simulink model "s_c_nbe_m32k"  (R2018a)
settings: Solver=VariableStepDiscrete  StartTime=0.0  StopTime=1000  RelTol=1e-3
undefined symbols (not defined in the file): fft_stages, n_taps, output_bits, pfb_coeff_gen_calc, xengbits
libraries: xbsIndex_r4 x23714, casper_library_misc x17, xps_library x4, casper_library_scopes x4, xbsReplacements_r4 x4
(part 25 of 171)

== system s_c_nbe_m32k/quant1 ==
  sync_in : Inport
  din : Inport  Port=2
  en : Inport  Port=3
  coeffs : Inport  Port=4
  Delay1 : xbsIndex_r4/Delay  rst=off  infoeditControl=Selection of Reset will increase slice count due to use of real FFs and instead of SRLs  en=off  latency=conv_latency  reg_retiming=on  dbl_ovrd=off  block_type=delay
  Delay2 : xbsIndex_r4/Delay  rst=off  infoeditControl=Selection of Reset will increase slice count due to use of real FFs and instead of SRLs  en=off  latency=conv_latency  reg_retiming=on  dbl_ovrd=off  block_type=delay
  Delay3 : xbsIndex_r4/Delay  rst=off  infoeditControl=Selection of Reset will increase slice count due to use of real FFs and instead of SRLs  en=off  latency=2  reg_retiming=on  dbl_ovrd=off  block_type=delay
  Delay4 : xbsIndex_r4/Delay  rst=off  infoeditControl=Selection of Reset will increase slice count due to use of real FFs and instead of SRLs  en=off  latency=2  reg_retiming=on  dbl_ovrd=off  block_type=delay
  Delay6 : xbsIndex_r4/Delay  rst=off  infoeditControl=Selection of Reset will increase slice count due to use of real FFs and instead of SRLs  en=off  latency=2  reg_retiming=on  dbl_ovrd=off  block_type=delay
  bus_constant : Subsystem  mask(bus_constant){values=repmat(-1+1/(2^dout_bin_pt), 1, 8), n_bits=dout_bit_width, bin_pts=dout_bin_pt, types=[1]}
      mask prompts: n_bits "bit widths"; bin_pts "binary points"; types "data type"
      mask help: Combine constants into a bus
      mask init:
      | bus_constant_init(gcb, ...
      |     'values', values, ...
      |     'n_bits', n_bits, ...
      |     'bin_pts', bin_pts, ...
      |     'types', types);
  bus_constant1 : Subsystem  mask(bus_constant){values=repmat(-1+1/(2^dout_bin_pt), 1, 8), n_bits=din_bit_width+coeff_bit_width+1, bin_pts=din_bin_pt+coeff_bin_pt, types=[1]}
      mask prompts: n_bits "bit widths"; bin_pts "binary points"; types "data type"
      mask help: Combine constants into a bus
      mask init:
      | bus_constant_init(gcb, ...
      |     'values', values, ...
      |     'n_bits', n_bits, ...
      |     'bin_pts', bin_pts, ...
      |     'types', types);
  bus_convert : Subsystem  Tag=cmac_delinked  mask(bus_convert){n_bits_in=repmat(din_bit_width+coeff_bit_width+1, 1, 8), bin_pt_in=din_bin_pt+coeff_bin_pt, cmplx=off, n_bits_out=8, bin_pt_out=7, quantization=2, overflow=1, csp_latency=conv_latency, of=on, misc=off}
      mask prompts: n_bits_in "input bit widths"; bin_pt_in "input binary points"; cmplx "input complex"; n_bits_out "output bit widths"; bin_pt_out "output binary points"; quantization "quantization strategy (Truncate=0, Round  (unbiased: +/- Inf)=1, Round (unbiased: Even Values)=2)"; overflow "overflow strategy (Wrap=0, Saturate=1, Flag as error=2)"; csp_latency "latency"; of "overflow indication"; misc "misc support"
      mask help: Convert components of busses
      mask init: same as s_c_nbe_m32k/cwg_cos/bus_convert
  bus_create : Subsystem  mask(bus_create){inputNum=2}
      mask prompts: inputNum "Number of inputs:"
      mask init:
      | bus_create_init(gcb,...
      |     'inputNum', inputNum);
  bus_expand1 : Subsystem  mask(bus_expand){mode=divisions of equal size, outputNum=2, outputWidth=1, outputBinaryPt=0, outputArithmeticType=2, show_format=off, outputToWorkspace=off, variablePrefix=out, outputToModelAsWell=on}
      mask prompts: outputNum "Number of outputs:"; outputWidth "Output width:"; outputBinaryPt "Output binary point position:"; outputArithmeticType "Output arithmetic type (ufix=0, fix=1, bool=2):"; show_format "Print format string?"; outputToWorkspace "Output to workspace?"; variablePrefix "Variable name prefix:"; outputToModelAsWell "Output to model as well?"
      mask help:
      | Expands a 'bus' made using a bus_create or Xilinx
      | concat block.
      | The input will be divided into the specified number
      | of outputs with the specified arithmetic types.
      | Divisions are made from most significant bit.
      mask init: same as s_c_nbe_m32k/bus_expand1
      settings: AttributesFormatString=2 outputs
      mask TypeOptions mode: divisions of equal size | divisions of arbitrary size
      mask Callback mode: bus_expand_callback();
      mask Callback outputWidth: bus_expand_callback();
      mask Callback outputToWorkspace: bus_expand_callback();
  bus_mult : Subsystem  mask(bus_mult){n_bits_a=repmat(din_bit_width, 1, 4), bin_pt_a=din_bin_pt, type_a=1, cmplx_a=on, n_bits_b=repmat(coeff_bit_width, 1, 4), bin_pt_b=coeff_bin_pt, type_b=1, cmplx_b=on, n_bits_out=din_bit_width+coeff_bit_width+1, bin_pt_out=din_bin_pt+coeff_bin_pt, type_out=1, quantization=0, overflow=0, mult_latency=3, add_latency=1, conv_latency=0, max_fanout=1, fan_latency=1, multiplier_implementation=behavioral HDL, misc=on}
      mask prompts: n_bits_a "a input bit widths"; bin_pt_a "a input binary points"; type_a "a input type (Unsigned=0, Signed=1)"; cmplx_a "a input complex"; n_bits_b "b input bit widths"; bin_pt_b "b input binary points"; type_b "b input type (Unsigned=0, Signed=1)"; cmplx_b "b input complex"; n_bits_out "output bit widths"; bin_pt_out "output binary points"; type_out "output type (Unsigned=0, Signed=1)"; quantization "quantization strategy (Truncate=0, Round  (unbiased: +/- Inf)=1)"; overflow "overflow strategy (Wrap=0, Saturate=1, Flag as error=2)"; mult_latency "multiplier latency"; add_latency "adder latency"; conv_latency "convert latency"; max_fanout "limit fanout to ?"; fan_latency "fanout register latency"; multiplier_implementation "multiplier implementation"; misc "misc support"
      mask help: Multiply components of two busses
      mask init: same as s_c_nbe_m32k/quant0/bus_mult
      mask TypeOptions multiplier_implementation: behavioral HDL | standard core | embedded multiplier core
  bus_mux : Subsystem  mask(bus_mux){n_inputs=2, n_bits=repmat(8, 1, 8), mux_latency=2, cmplx=off, misc=off}
      mask prompts: n_inputs "number of inputs"; n_bits "input bit widths"; mux_latency "mux latency"; cmplx "complex data"; misc "misc support"
      mask help: Mux components of bus
      mask init:
      | bus_mux_init(gcb, ...
      |     'n_inputs', n_inputs, ...
      |     'n_bits', n_bits, ...
      |     'cmplx', cmplx, ...
      |     'misc', misc, ...
      |     'mux_latency', mux_latency);
  bus_relational : Subsystem  Tag=cmac_delinked  mask(bus_relational){n_bits_a=repmat(din_bit_width+coeff_bit_width+1, 1, 8), bin_pt_a=din_bin_pt+coeff_bin_pt, type_a=1, n_bits_b=repmat(din_bit_width+coeff_bit_width+1, 1, 8), bin_pt_b=din_bin_pt+coeff_bin_pt, type_b=1, en=off, misc=off, mode=a<b, csp_latency=conv_latency}
      mask prompts: n_bits_a "a input bit widths"; bin_pt_a "a input binary points"; type_a "a input type (Unsigned=0, Signed=1)"; n_bits_b "b input bit widths"; bin_pt_b "b input binary points"; type_b "b input type (Unsigned=0, Signed=1)"; en "en port"; misc "misc support"; mode "comparison:"; csp_latency "latency"
      mask help: Find the relational product of two busses
      mask init: same as s_c_nbe_m32k/quant0/bus_relational
      mask TypeOptions mode: a=b | a!=b | a<b | a>b | a<=b | a>=b
  pipeline1 : Subsystem  Tag=cmac_delinked  mask(pipeline){csp_latency=2}
      mask prompts: csp_latency "Latency"
      mask help:
      | An explicitly laid-out delay line to avoid mapping to SRL16s
      | for use in pipelining to help achieve timing closure.
      mask init:
      | pipeline_init(gcb,'latency',csp_latency);
      settings: AttributesFormatString=Latency = %<latency>
      mask Display:
      | port_label('input', 1, 'd');
      | port_label('output', 1, 'q');
      | disp(['Z^-', num2str(csp_latency)]);
  pipeline10 : Subsystem  Tag=cmac_delinked  mask(pipeline){csp_latency=2}
      mask prompts: csp_latency "Latency"
      mask help:
      | An explicitly laid-out delay line to avoid mapping to SRL16s
      | for use in pipelining to help achieve timing closure.
      mask init:
      | pipeline_init(gcb,'latency',csp_latency);
      settings: AttributesFormatString=Latency = %<latency>
      mask Display:
      | port_label('input', 1, 'd');
      | port_label('output', 1, 'q');
      | disp(['Z^-', num2str(csp_latency)]);
  pipeline2 : Subsystem  Tag=cmac_delinked  mask(pipeline){csp_latency=2}
      mask prompts: csp_latency "Latency"
      mask help:
      | An explicitly laid-out delay line to avoid mapping to SRL16s
      | for use in pipelining to help achieve timing closure.
      mask init:
      | pipeline_init(gcb,'latency',csp_latency);
      settings: AttributesFormatString=Latency = %<latency>
      mask Display:
      | port_label('input', 1, 'd');
      | port_label('output', 1, 'q');
      | disp(['Z^-', num2str(csp_latency)]);
  pipeline3 : Subsystem  Tag=cmac_delinked  mask(pipeline){csp_latency=2}
      mask prompts: csp_latency "Latency"
      mask help:
      | An explicitly laid-out delay line to avoid mapping to SRL16s
      | for use in pipelining to help achieve timing closure.
      mask init:
      | pipeline_init(gcb,'latency',csp_latency);
      settings: AttributesFormatString=Latency = %<latency>
      mask Display:
      | port_label('input', 1, 'd');
      | port_label('output', 1, 'q');
      | disp(['Z^-', num2str(csp_latency)]);
  pipeline4 : Subsystem  Tag=cmac_delinked  mask(pipeline){csp_latency=2}
      mask prompts: csp_latency "Latency"
      mask help:
      | An explicitly laid-out delay line to avoid mapping to SRL16s
      | for use in pipelining to help achieve timing closure.
      mask init:
      | pipeline_init(gcb,'latency',csp_latency);
      settings: AttributesFormatString=Latency = %<latency>
      mask Display:
      | port_label('input', 1, 'd');
      | port_label('output', 1, 'q');
      | disp(['Z^-', num2str(csp_latency)]);
  pipeline45 : Subsystem  Tag=cmac_delinked  mask(pipeline){csp_latency=2}
      mask prompts: csp_latency "Latency"
      mask help:
      | An explicitly laid-out delay line to avoid mapping to SRL16s
      | for use in pipelining to help achieve timing closure.
      mask init:
      | pipeline_init(gcb,'latency',csp_latency);
      settings: AttributesFormatString=Latency = %<latency>
      mask Display:
      | port_label('input', 1, 'd');
      | port_label('output', 1, 'q');
      | disp(['Z^-', num2str(csp_latency)]);
  pipeline5 : Subsystem  Tag=cmac_delinked  mask(pipeline){csp_latency=2}
      mask prompts: csp_latency "Latency"
      mask help:
      | An explicitly laid-out delay line to avoid mapping to SRL16s
      | for use in pipelining to help achieve timing closure.
      mask init:
      | pipeline_init(gcb,'latency',csp_latency);
      settings: AttributesFormatString=Latency = %<latency>
      mask Display:
      | port_label('input', 1, 'd');
      | port_label('output', 1, 'q');
      | disp(['Z^-', num2str(csp_latency)]);
  pipeline6 : Subsystem  Tag=cmac_delinked  mask(pipeline){csp_latency=2}
      mask prompts: csp_latency "Latency"
      mask help:
      | An explicitly laid-out delay line to avoid mapping to SRL16s
      | for use in pipelining to help achieve timing closure.
      mask init:
      | pipeline_init(gcb,'latency',csp_latency);
      settings: AttributesFormatString=Latency = %<latency>
      mask Display:
      | port_label('input', 1, 'd');
      | port_label('output', 1, 'q');
      | disp(['Z^-', num2str(csp_latency)]);
  pipeline7 : Subsystem  Tag=cmac_delinked  mask(pipeline){csp_latency=2}
      mask prompts: csp_latency "Latency"
      mask help:
      | An explicitly laid-out delay line to avoid mapping to SRL16s
      | for use in pipelining to help achieve timing closure.
      mask init:
      | pipeline_init(gcb,'latency',csp_latency);
      settings: AttributesFormatString=Latency = %<latency>
      mask Display:
      | port_label('input', 1, 'd');
      | port_label('output', 1, 'q');
      | disp(['Z^-', num2str(csp_latency)]);
  pipeline8 : Subsystem  Tag=cmac_delinked  mask(pipeline){csp_latency=2}
      mask prompts: csp_latency "Latency"
      mask help:
      | An explicitly laid-out delay line to avoid mapping to SRL16s
      | for use in pipelining to help achieve timing closure.
      mask init:
      | pipeline_init(gcb,'latency',csp_latency);
      settings: AttributesFormatString=Latency = %<latency>
      mask Display:
      | port_label('input', 1, 'd');
      | port_label('output', 1, 'q');
      | disp(['Z^-', num2str(csp_latency)]);
  pipeline9 : Subsystem  Tag=cmac_delinked  mask(pipeline){csp_latency=2}
      mask prompts: csp_latency "Latency"
      mask help:
      | An explicitly laid-out delay line to avoid mapping to SRL16s
      | for use in pipelining to help achieve timing closure.
      mask init:
      | pipeline_init(gcb,'latency',csp_latency);
      settings: AttributesFormatString=Latency = %<latency>
      mask Display:
      | port_label('input', 1, 'd');
      | port_label('output', 1, 'q');
      | disp(['Z^-', num2str(csp_latency)]);
  sync_out : Outport
  dout : Outport  Port=2
  dvalid : Outport  Port=3
  of : Outport  Port=4
  wires:
  pipeline10/1(q) -> dvalid/1
  pipeline9/1(q) -> sync_out/1
  pipeline8/1(q) -> of/1
  pipeline7/1(q) -> dout/1
  pipeline6/1(q) -> bus_expand1/1(bus_in)
  pipeline5/1(q) -> bus_convert/1(din)
  pipeline4/1(q) -> bus_relational/1(a)
  pipeline3/1(q) -> bus_create/2(in2)
  pipeline2/1(q) -> bus_create/1(in1)
  pipeline1/1(q) -> bus_mult/2(b)
  pipeline45/1(q) -> bus_mult/1(a)
  Delay4/1 -> pipeline8/1(d)
  bus_convert/2(overflow) -> Delay4/1
  bus_mux/1(out) -> pipeline7/1(d)
  bus_constant1/1(dout) -> bus_relational/2(b)
  bus_constant/1(dout) -> bus_mux/3(d1)
  bus_convert/1(dout) -> bus_mux/2(d0)
  bus_relational/1(a<b) -> bus_mux/1(sel)
  Delay3/1 -> pipeline10/1(d)
  bus_expand1/2(lsb_out1) -> Delay1/1
  Delay1/1 -> Delay3/1
  bus_expand1/1(msb_out2) -> Delay2/1
  bus_mult/2(misco) -> pipeline6/1(d)
  bus_mult/1(a*b) -> pipeline4/1(d), pipeline5/1(d)
  bus_create/1(bus_out) -> bus_mult/3(misci)
  en/1 -> pipeline3/1(d)
  sync_in/1 -> pipeline2/1(d)
  coeffs/1 -> pipeline1/1(d)
  din/1 -> pipeline45/1(d)
  Delay6/1 -> pipeline9/1(d)
  Delay2/1 -> Delay6/1

== system s_c_nbe_m32k/quant_pwr0 ==
  out_reg : Inport
  assert_reg : xbsIndex_r4/Assert  assert_type=on  type_source=Explicitly  gui_display_data_type=Fixed-point  arith_type=Unsigned  n_bits=32  bin_pt=31  preci_type=Single  exp_width=8  frac_width=24  assert_rate=off  rate_source=Explicitly  period=1  output_port=on  block_type=assert
  cast_gw : xbsIndex_r4/Convert  gui_display_data_type=Fixed-point  arith_type=Unsigned  n_bits=32  bin_pt=0  float_type=Single  exp_bits=8  fraction_bits=24  quantization=Truncate  overflow=Wrap  en=off  latency=1  pipeline=off  dbl_ovrd=off  block_type=convert
  io_delay : xbsIndex_r4/Delay  rst=off  infoeditControl=Selection of Reset will increase slice count due to use of real FFs and instead of SRLs  en=off  latency=0  reg_retiming=on  dbl_ovrd=off  block_type=delay
  reint1 : xbsIndex_r4/Reinterpret  force_arith_type=on  arith_type=Unsigned  force_bin_pt=on  bin_pt=0  block_type=reinterpret
  s_c_nbe_m32k_v9_quant_pwr0_user_data_in : xbsIndex_r4/Gateway Out  inherit_from_input=off  hdl_port=on  rows=1  columns=1  UseAsDAC=off  DACChannel='1'  interface=None  automatic_assignment=on  address_offset=hex2dec('00')  intf_name=''  intf_description=''  timing_constraint=None  locs_specified=off  LOCs={}  io_standard={}  block_type=gatewayout
  sim_out : Terminator
  wires:
  io_delay/1 -> cast_gw/1
  cast_gw/1 -> s_c_nbe_m32k_v9_quant_pwr0_user_data_in/1
  s_c_nbe_m32k_v9_quant_pwr0_user_data_in/1 -> sim_out/1
  out_reg/1 -> assert_reg/1
  assert_reg/1 -> reint1/1
  reint1/1 -> io_delay/1

== system s_c_nbe_m32k/quant_pwr1 ==
  out_reg : Inport
  assert_reg : xbsIndex_r4/Assert  assert_type=on  type_source=Explicitly  gui_display_data_type=Fixed-point  arith_type=Unsigned  n_bits=32  bin_pt=31  preci_type=Single  exp_width=8  frac_width=24  assert_rate=off  rate_source=Explicitly  period=1  output_port=on  block_type=assert
  cast_gw : xbsIndex_r4/Convert  gui_display_data_type=Fixed-point  arith_type=Unsigned  n_bits=32  bin_pt=0  float_type=Single  exp_bits=8  fraction_bits=24  quantization=Truncate  overflow=Wrap  en=off  latency=1  pipeline=off  dbl_ovrd=off  block_type=convert
  io_delay : xbsIndex_r4/Delay  rst=off  infoeditControl=Selection of Reset will increase slice count due to use of real FFs and instead of SRLs  en=off  latency=0  reg_retiming=on  dbl_ovrd=off  block_type=delay
  reint1 : xbsIndex_r4/Reinterpret  force_arith_type=on  arith_type=Unsigned  force_bin_pt=on  bin_pt=0  block_type=reinterpret
  s_c_nbe_m32k_v9_quant_pwr1_user_data_in : xbsIndex_r4/Gateway Out  inherit_from_input=off  hdl_port=on  rows=1  columns=1  UseAsDAC=off  DACChannel='1'  interface=None  automatic_assignment=on  address_offset=hex2dec('00')  intf_name=''  intf_description=''  timing_constraint=None  locs_specified=off  LOCs={}  io_standard={}  block_type=gatewayout
  sim_out : Terminator
  wires:
  io_delay/1 -> cast_gw/1
  cast_gw/1 -> s_c_nbe_m32k_v9_quant_pwr1_user_data_in/1
  s_c_nbe_m32k_v9_quant_pwr1_user_data_in/1 -> sim_out/1
  out_reg/1 -> assert_reg/1
  assert_reg/1 -> reint1/1
  reint1/1 -> io_delay/1

== system s_c_nbe_m32k/quant_snap_ctrl ==
  sim_1 : Inport
  sim_2 : Inport  Port=2
  convert1_1 : DataTypeConversion  OutDataTypeStr=fixdt('ufix1_En0')  LockScale=on
  convert1_2 : DataTypeConversion  OutDataTypeStr=fixdt('ufix31_En0')  LockScale=on
  convert2_1 : DataTypeConversion  OutDataTypeStr=fixdt('ufix1_En0')  ConvertRealWorld=Stored Integer (SI)  LockScale=on
  convert2_2 : DataTypeConversion  OutDataTypeStr=fixdt('ufix31_En0')  ConvertRealWorld=Stored Integer (SI)  LockScale=on
  gain_1 : Gain  Gain=2147483648
  gain_2 : Gain
  io_delay : xbsIndex_r4/Delay  rst=off  infoeditControl=Selection of Reset will increase slice count due to use of real FFs and instead of SRLs  en=off  latency=0  reg_retiming=on  dbl_ovrd=off  block_type=delay
  reint2 : xbsIndex_r4/Reinterpret  force_arith_type=on  arith_type=Unsigned  force_bin_pt=on  bin_pt=0  block_type=reinterpret
  s_c_nbe_m32k_v9_quant_snap_ctrl_user_data_out : xbsIndex_r4/Gateway In  gui_display_data_type=Fixed-point  arith_type=Unsigned  n_bits=32  bin_pt=0  preci_type=Single  exp_width=8  frac_width=24  rows=1  columns=1  quantization="Round  (unbiased: +/- Inf)"  overflow=Saturate  period=1  UseAsADC=off  ADCChannel='1'  interface=None  automatic_assignment=on  address_offset=hex2dec('00')  intf_name=''  intf_description=''  default_value=0  timing_constraint=None  locs_specified=off  LOCs={}  io_standard={}  inherit_from_input=off  hdl_port=on  dbl_ovrd=off  block_type=gatewayin
  sim_add : Sum  OutDataTypeStr=uint32
  slice_channel_select : xbsIndex_r4/Slice  nbits=31  boolean_output=off  mode=Lower Bit Location + Width  bit1=0  base1=MSB of Input  bit0=0  base0=LSB of Input  dbl_ovrd=off  block_type=slice
  slice_single_channel : xbsIndex_r4/Slice  nbits=1  boolean_output=on  mode=Lower Bit Location + Width  bit1=0  base1=MSB of Input  bit0=31  base0=LSB of Input  dbl_ovrd=off  block_type=slice
  in_single_channel : Outport
  in_channel_select : Outport  Port=2
  wires:
  s_c_nbe_m32k_v9_quant_snap_ctrl_user_data_out/1 -> io_delay/1
  sim_add/1 -> s_c_nbe_m32k_v9_quant_snap_ctrl_user_data_out/1
  sim_1/1 -> convert1_1/1
  convert1_1/1 -> convert2_1/1
  convert2_1/1 -> gain_1/1
  gain_1/1 -> sim_add/1
  io_delay/1 -> slice_single_channel/1, slice_channel_select/1
  slice_single_channel/1 -> in_single_channel/1
  sim_2/1 -> convert1_2/1
  convert1_2/1 -> convert2_2/1
  convert2_2/1 -> gain_2/1
  gain_2/1 -> sim_add/2
  slice_channel_select/1 -> reint2/1
  reint2/1 -> in_channel_select/1

== system s_c_nbe_m32k/quant_snap_filter0 ==
  note: This block filters out a single channel
      | from the quantiser so that if you want to get
      | a time-series of them in the snap instead of
      | a spectrum, you can do so.
  sync_in : Inport
  data_valid_in : Inport  Port=2
  data_in : Inport  Port=3
  packet_sync_in : Inport  Port=4
  single_channel_enable : Inport  Port=5
  channel_select : Inport  Port=6
  Counter : xbsIndex_r4/Counter  cnt_type=Free Running  cnt_to=4095  operation=Up  start_count=0  cnt_by_val=1  arith_type=Unsigned  n_bits=fft_stages - 3  bin_pt=0  load_pin=off  rst=on  en=on  explicit_period=on  period=1  use_behavioral_HDL=off  implementation=Fabric  dbl_ovrd=off  block_type=counter
  Delay : xbsIndex_r4/Delay  rst=off  infoeditControl=Selection of Reset will increase slice count due to use of real FFs and instead of SRLs  en=off  latency=1  reg_retiming=off  dbl_ovrd=off  block_type=delay
      settings: infoedit=Hardware notes: A delay line is a chain, each link of which is an SRL16 or SRL32 followed by a flip-flop.
  Delay1 : xbsIndex_r4/Delay  rst=off  infoeditControl=Selection of Reset will increase slice count due to use of real FFs and instead of SRLs  en=off  latency=1  reg_retiming=off  dbl_ovrd=off  block_type=delay
      settings: infoedit=Hardware notes: A delay line is a chain, each link of which is an SRL16 or SRL32 followed by a flip-flop.
  Mux1 : xbsIndex_r4/Mux  inputs=2  en=off  latency=3  precision=Full  arith_type=Unsigned  n_bits=16  bin_pt=14  quantization=Truncate  overflow=Wrap  dbl_ovrd=off  block_type=mux
  Relational : xbsIndex_r4/Relational  mode=a=b  op_type=Bool  en=off  latency=0  dbl_ovrd=off  block_type=relational
  data_valid_out : Outport
  data_out : Outport  Port=2
  packet_sync_out : Outport  Port=3
  wires:
  [packet_sync] -> Delay1/1
  Delay/1 -> data_out/1
  data_valid_in/1 -> [data_valid]
  [sync_in] -> Counter/1
  Mux1/1 -> data_valid_out/1
  data_in/1 -> [data]
  [data_valid] -> Mux1/2
  Relational/1 -> [selected_channel_active]
  Counter/1 -> Relational/1
  sync_in/1 -> [sync_in]
  [selected_channel_active] -> Mux1/3
  packet_sync_in/1 -> [packet_sync]
  [data] -> Delay/1
  [channel_select] -> Relational/2
  Delay1/1 -> packet_sync_out/1
  single_channel_enable/1 -> [single_channel_enable]
  [data_valid] -> Counter/2
  [single_channel_enable] -> Mux1/1
  channel_select/1 -> [channel_select]

== system s_c_nbe_m32k/quant_snap_filter1 ==
  note: This block filters out a single channel
      | from the quantiser so that if you want to get
      | a time-series of them in the snap instead of
      | a spectrum, you can do so.
  sync_in : Inport
  data_valid_in : Inport  Port=2
  data_in : Inport  Port=3
  packet_sync_in : Inport  Port=4
  single_channel_enable : Inport  Port=5
  channel_select : Inport  Port=6
  Counter : xbsIndex_r4/Counter  cnt_type=Free Running  cnt_to=4095  operation=Up  start_count=0  cnt_by_val=1  arith_type=Unsigned  n_bits=fft_stages - 3  bin_pt=0  load_pin=off  rst=on  en=on  explicit_period=on  period=1  use_behavioral_HDL=off  implementation=Fabric  dbl_ovrd=off  block_type=counter
  Delay : xbsIndex_r4/Delay  rst=off  infoeditControl=Selection of Reset will increase slice count due to use of real FFs and instead of SRLs  en=off  latency=1  reg_retiming=off  dbl_ovrd=off  block_type=delay
      settings: infoedit=Hardware notes: A delay line is a chain, each link of which is an SRL16 or SRL32 followed by a flip-flop.
  Delay1 : xbsIndex_r4/Delay  rst=off  infoeditControl=Selection of Reset will increase slice count due to use of real FFs and instead of SRLs  en=off  latency=1  reg_retiming=off  dbl_ovrd=off  block_type=delay
      settings: infoedit=Hardware notes: A delay line is a chain, each link of which is an SRL16 or SRL32 followed by a flip-flop.
  Mux1 : xbsIndex_r4/Mux  inputs=2  en=off  latency=3  precision=Full  arith_type=Unsigned  n_bits=16  bin_pt=14  quantization=Truncate  overflow=Wrap  dbl_ovrd=off  block_type=mux
  Relational : xbsIndex_r4/Relational  mode=a=b  op_type=Bool  en=off  latency=0  dbl_ovrd=off  block_type=relational
  data_valid_out : Outport
  data_out : Outport  Port=2
  packet_sync_out : Outport  Port=3
  wires:
  channel_select/1 -> [channel_select]
  [single_channel_enable] -> Mux1/1
  [data_valid] -> Counter/2
  single_channel_enable/1 -> [single_channel_enable]
  Delay1/1 -> packet_sync_out/1
  [channel_select] -> Relational/2
  [data] -> Delay/1
  packet_sync_in/1 -> [packet_sync]
  [selected_channel_active] -> Mux1/3
  sync_in/1 -> [sync_in]
  Counter/1 -> Relational/1
  Relational/1 -> [selected_channel_active]
  [data_valid] -> Mux1/2
  data_in/1 -> [data]
  Mux1/1 -> data_valid_out/1
  [sync_in] -> Counter/1
  data_valid_in/1 -> [data_valid]
  Delay/1 -> data_out/1
  [packet_sync] -> Delay1/1

== system s_c_nbe_m32k/quant_status ==
  out_pol0_or_cnt : Inport
  out_pol1_or_cnt : Inport  Port=2
  assert_pol0_or_cnt : xbsIndex_r4/Assert  assert_type=on  type_source=Explicitly  gui_display_data_type=Fixed-point  arith_type=Unsigned  n_bits=6  bin_pt=0  preci_type=Single  exp_width=8  frac_width=24  assert_rate=off  rate_source=Explicitly  period=1  output_port=on  block_type=assert
  assert_pol1_or_cnt : xbsIndex_r4/Assert  assert_type=on  type_source=Explicitly  gui_display_data_type=Fixed-point  arith_type=Unsigned  n_bits=6  bin_pt=0  preci_type=Single  exp_width=8  frac_width=24  assert_rate=off  rate_source=Explicitly  period=1  output_port=on  block_type=assert
  cast_gw : xbsIndex_r4/Convert  gui_display_data_type=Fixed-point  arith_type=Unsigned  n_bits=32  bin_pt=0  float_type=Single  exp_bits=8  fraction_bits=24  quantization=Truncate  overflow=Wrap  en=off  latency=1  pipeline=off  dbl_ovrd=off  block_type=convert
  concatenate : xbsIndex_r4/Concat  num_inputs=2  dbl_ovrd=off  block_type=concat
  io_delay : xbsIndex_r4/Delay  rst=off  infoeditControl=Selection of Reset will increase slice count due to use of real FFs and instead of SRLs  en=off  latency=0  reg_retiming=on  dbl_ovrd=off  block_type=delay
  reint1 : xbsIndex_r4/Reinterpret  force_arith_type=on  arith_type=Unsigned  force_bin_pt=on  bin_pt=0  block_type=reinterpret
  reint2 : xbsIndex_r4/Reinterpret  force_arith_type=on  arith_type=Unsigned  force_bin_pt=on  bin_pt=0  block_type=reinterpret
  s_c_nbe_m32k_v9_quant_status_user_data_in : xbsIndex_r4/Gateway Out  inherit_from_input=off  hdl_port=on  rows=1  columns=1  UseAsDAC=off  DACChannel='1'  interface=None  automatic_assignment=on  address_offset=hex2dec('00')  intf_name=''  intf_description=''  timing_constraint=None  locs_specified=off  LOCs={}  io_standard={}  block_type=gatewayout
  sim_out : Terminator
  wires:
  concatenate/1 -> io_delay/1
  io_delay/1 -> cast_gw/1
  cast_gw/1 -> s_c_nbe_m32k_v9_quant_status_user_data_in/1
  s_c_nbe_m32k_v9_quant_status_user_data_in/1 -> sim_out/1
  out_pol0_or_cnt/1 -> assert_pol0_or_cnt/1
  assert_pol0_or_cnt/1 -> reint1/1
  reint1/1 -> concatenate/1
  out_pol1_or_cnt/1 -> assert_pol1_or_cnt/1
  assert_pol1_or_cnt/1 -> reint2/1
  reint2/1 -> concatenate/2

== system s_c_nbe_m32k/quant_sync_cnt ==
  out_reg : Inport
  assert_reg : xbsIndex_r4/Assert  assert_type=on  type_source=Explicitly  gui_display_data_type=Fixed-point  arith_type=Unsigned  n_bits=8  bin_pt=0  preci_type=Single  exp_width=8  frac_width=24  assert_rate=off  rate_source=Explicitly  period=1  output_port=on  block_type=assert
  cast_gw : xbsIndex_r4/Convert  gui_display_data_type=Fixed-point  arith_type=Unsigned  n_bits=32  bin_pt=0  float_type=Single  exp_bits=8  fraction_bits=24  quantization=Truncate  overflow=Wrap  en=off  latency=1  pipeline=off  dbl_ovrd=off  block_type=convert
  io_delay : xbsIndex_r4/Delay  rst=off  infoeditControl=Selection of Reset will increase slice count due to use of real FFs and instead of SRLs  en=off  latency=0  reg_retiming=on  dbl_ovrd=off  block_type=delay
  reint1 : xbsIndex_r4/Reinterpret  force_arith_type=on  arith_type=Unsigned  force_bin_pt=on  bin_pt=0  block_type=reinterpret
  s_c_nbe_m32k_v9_quant_sync_cnt_user_data_in : xbsIndex_r4/Gateway Out  inherit_from_input=off  hdl_port=on  rows=1  columns=1  UseAsDAC=off  DACChannel='1'  interface=None  automatic_assignment=on  address_offset=hex2dec('00')  intf_name=''  intf_description=''  timing_constraint=None  locs_specified=off  LOCs={}  io_standard={}  block_type=gatewayout
  sim_out : Terminator
  wires:
  io_delay/1 -> cast_gw/1
  cast_gw/1 -> s_c_nbe_m32k_v9_quant_sync_cnt_user_data_in/1
  s_c_nbe_m32k_v9_quant_sync_cnt_user_data_in/1 -> sim_out/1
  out_reg/1 -> assert_reg/1
  assert_reg/1 -> reint1/1
  reint1/1 -> io_delay/1

== system s_c_nbe_m32k/re_im_interleave ==
  In1 : Inport
  In2 : Inport  Port=2
  Concat{1..8} (8 alike) : xbsIndex_r4/Concat  num_inputs=2  dbl_ovrd=off  block_type=concat
  Concat9 : xbsIndex_r4/Concat  num_inputs=8  dbl_ovrd=off  block_type=concat
  Reinterpret{,1..15} (16 alike) : xbsIndex_r4/Reinterpret  force_arith_type=on  arith_type=Unsigned  force_bin_pt=on  bin_pt=0  block_type=reinterpret
  bus_expand6 : Subsystem  mask(bus_expand){mode=divisions of equal size, outputNum=8, outputWidth=18, outputBinaryPt=17, outputArithmeticType=1, show_format=off, outputToWorkspace=off, variablePrefix=out, outputToModelAsWell=on}
      mask prompts: outputNum "Number of outputs:"; outputWidth "Output width:"; outputBinaryPt "Output binary point position:"; outputArithmeticType "Output arithmetic type (ufix=0, fix=1, bool=2):"; show_format "Print format string?"; outputToWorkspace "Output to workspace?"; variablePrefix "Variable name prefix:"; outputToModelAsWell "Output to model as well?"
      mask help:
      | Expands a 'bus' made using a bus_create or Xilinx
      | concat block.
      | The input will be divided into the specified number
      | of outputs with the specified arithmetic types.
      | Divisions are made from most significant bit.
      mask init: same as s_c_nbe_m32k/bus_expand1
      settings: AttributesFormatString=8 outputs
      mask TypeOptions mode: divisions of equal size | divisions of arbitrary size
      mask Callback mode: bus_expand_callback();
      mask Callback outputWidth: bus_expand_callback();
      mask Callback outputToWorkspace: bus_expand_callback();
  bus_expand7 : Subsystem  mask(bus_expand){mode=divisions of equal size, outputNum=8, outputWidth=18, outputBinaryPt=17, outputArithmeticType=1, show_format=off, outputToWorkspace=off, variablePrefix=out, outputToModelAsWell=on}
      mask prompts: outputNum "Number of outputs:"; outputWidth "Output width:"; outputBinaryPt "Output binary point position:"; outputArithmeticType "Output arithmetic type (ufix=0, fix=1, bool=2):"; show_format "Print format string?"; outputToWorkspace "Output to workspace?"; variablePrefix "Variable name prefix:"; outputToModelAsWell "Output to model as well?"
      mask help:
      | Expands a 'bus' made using a bus_create or Xilinx
      | concat block.
      | The input will be divided into the specified number
      | of outputs with the specified arithmetic types.
      | Divisions are made from most significant bit.
      mask init: same as s_c_nbe_m32k/bus_expand1
      settings: AttributesFormatString=8 outputs
      mask TypeOptions mode: divisions of equal size | divisions of arbitrary size
      mask Callback mode: bus_expand_callback();
      mask Callback outputWidth: bus_expand_callback();
      mask Callback outputToWorkspace: bus_expand_callback();
  Out1 : Outport
  wires:
  In2/1 -> bus_expand7/1(bus_in)
  Concat2/1 -> Concat9/2
  Concat1/1 -> Concat9/1
  bus_expand6/7(out2) -> Reinterpret6/1
  Concat7/1 -> Concat9/7
  bus_expand7/4(out5) -> Reinterpret11/1
  bus_expand6/1(msb_out8) -> Reinterpret/1
  Concat6/1 -> Concat9/6
  bus_expand6/4(out5) -> Reinterpret3/1
  bus_expand7/8(lsb_out1) -> Reinterpret15/1
  In1/1 -> bus_expand6/1(bus_in)
  bus_expand7/3(out6) -> Reinterpret10/1
  bus_expand6/6(out3) -> Reinterpret5/1
  bus_expand7/1(msb_out8) -> Reinterpret8/1
  bus_expand6/2(out7) -> Reinterpret1/1
  bus_expand6/8(lsb_out1) -> Reinterpret7/1
  Concat5/1 -> Concat9/5
  bus_expand6/3(out6) -> Reinterpret2/1
  bus_expand7/5(out4) -> Reinterpret12/1
  Concat9/1 -> Out1/1
  bus_expand7/2(out7) -> Reinterpret9/1
  Concat8/1 -> Concat9/8
  bus_expand6/5(out4) -> Reinterpret4/1
  Concat3/1 -> Concat9/3
  bus_expand7/6(out3) -> Reinterpret13/1
  Concat4/1 -> Concat9/4
  bus_expand7/7(out2) -> Reinterpret14/1
  Reinterpret/1 -> Concat1/1
  Reinterpret1/1 -> Concat2/1
  Reinterpret2/1 -> Concat3/1
  Reinterpret3/1 -> Concat4/1
  Reinterpret4/1 -> Concat5/1
  Reinterpret5/1 -> Concat6/1
  Reinterpret6/1 -> Concat7/1
  Reinterpret7/1 -> Concat8/1
  Reinterpret9/1 -> Concat2/2
  Reinterpret14/1 -> Concat7/2
  Reinterpret15/1 -> Concat8/2
  Reinterpret10/1 -> Concat3/2
  Reinterpret13/1 -> Concat6/2
  Reinterpret11/1 -> Concat4/2
  Reinterpret8/1 -> Concat1/2
  Reinterpret12/1 -> Concat5/2

== system s_c_nbe_m32k/reorder_status ==
  out_timestep_err_cnt : Inport
  out_receive_err_cnt : Inport  Port=2
  out_discard_cnt : Inport  Port=3
  out_relock_err_cnt : Inport  Port=4
  out_overflow_err_cnt : Inport  Port=5
  out_dv_cnt : Inport  Port=6
  assert_discard_cnt : xbsIndex_r4/Assert  assert_type=on  type_source=Explicitly  gui_display_data_type=Fixed-point  arith_type=Unsigned  n_bits=5  bin_pt=0  preci_type=Single  exp_width=8  frac_width=24  assert_rate=off  rate_source=Explicitly  period=1  output_port=on  block_type=assert
  assert_dv_cnt : xbsIndex_r4/Assert  assert_type=on  type_source=Explicitly  gui_display_data_type=Fixed-point  arith_type=Unsigned  n_bits=5  bin_pt=0  preci_type=Single  exp_width=8  frac_width=24  assert_rate=off  rate_source=Explicitly  period=1  output_port=on  block_type=assert
  assert_overflow_err_cnt : xbsIndex_r4/Assert  assert_type=on  type_source=Explicitly  gui_display_data_type=Fixed-point  arith_type=Unsigned  n_bits=5  bin_pt=0  preci_type=Single  exp_width=8  frac_width=24  assert_rate=off  rate_source=Explicitly  period=1  output_port=on  block_type=assert
  assert_receive_err_cnt : xbsIndex_r4/Assert  assert_type=on  type_source=Explicitly  gui_display_data_type=Fixed-point  arith_type=Unsigned  n_bits=5  bin_pt=0  preci_type=Single  exp_width=8  frac_width=24  assert_rate=off  rate_source=Explicitly  period=1  output_port=on  block_type=assert
  assert_relock_err_cnt : xbsIndex_r4/Assert  assert_type=on  type_source=Explicitly  gui_display_data_type=Fixed-point  arith_type=Unsigned  n_bits=5  bin_pt=0  preci_type=Single  exp_width=8  frac_width=24  assert_rate=off  rate_source=Explicitly  period=1  output_port=on  block_type=assert
  assert_timestep_err_cnt : xbsIndex_r4/Assert  assert_type=on  type_source=Explicitly  gui_display_data_type=Fixed-point  arith_type=Unsigned  n_bits=5  bin_pt=0  preci_type=Single  exp_width=8  frac_width=24  assert_rate=off  rate_source=Explicitly  period=1  output_port=on  block_type=assert
  cast_gw : xbsIndex_r4/Convert  gui_display_data_type=Fixed-point  arith_type=Unsigned  n_bits=32  bin_pt=0  float_type=Single  exp_bits=8  fraction_bits=24  quantization=Truncate  overflow=Wrap  en=off  latency=1  pipeline=off  dbl_ovrd=off  block_type=convert
  concatenate : xbsIndex_r4/Concat  num_inputs=6  dbl_ovrd=off  block_type=concat
  io_delay : xbsIndex_r4/Delay  rst=off  infoeditControl=Selection of Reset will increase slice count due to use of real FFs and instead of SRLs  en=off  latency=0  reg_retiming=on  dbl_ovrd=off  block_type=delay
  reint{1..6} (6 alike) : xbsIndex_r4/Reinterpret  force_arith_type=on  arith_type=Unsigned  force_bin_pt=on  bin_pt=0  block_type=reinterpret
  s_c_nbe_m32k_v9_reorder_status_user_data_in : xbsIndex_r4/Gateway Out  inherit_from_input=off  hdl_port=on  rows=1  columns=1  UseAsDAC=off  DACChannel='1'  interface=None  automatic_assignment=on  address_offset=hex2dec('00')  intf_name=''  intf_description=''  timing_constraint=None  locs_specified=off  LOCs={}  io_standard={}  block_type=gatewayout
  sim_out : Terminator
  wires:
  concatenate/1 -> io_delay/1
  io_delay/1 -> cast_gw/1
  cast_gw/1 -> s_c_nbe_m32k_v9_reorder_status_user_data_in/1
  s_c_nbe_m32k_v9_reorder_status_user_data_in/1 -> sim_out/1
  out_timestep_err_cnt/1 -> assert_timestep_err_cnt/1
  assert_timestep_err_cnt/1 -> reint1/1
  reint1/1 -> concatenate/1
  out_receive_err_cnt/1 -> assert_receive_err_cnt/1
  assert_receive_err_cnt/1 -> reint2/1
  reint2/1 -> concatenate/2
  out_discard_cnt/1 -> assert_discard_cnt/1
  assert_discard_cnt/1 -> reint3/1
  reint3/1 -> concatenate/3
  out_relock_err_cnt/1 -> assert_relock_err_cnt/1
  assert_relock_err_cnt/1 -> reint4/1
  reint4/1 -> concatenate/4
  out_overflow_err_cnt/1 -> assert_overflow_err_cnt/1
  assert_overflow_err_cnt/1 -> reint5/1
  reint5/1 -> concatenate/5
  out_dv_cnt/1 -> assert_dv_cnt/1
  assert_dv_cnt/1 -> reint6/1
  reint6/1 -> concatenate/6

== system s_c_nbe_m32k/reorder_status1 ==
  out_dv_per_sec : Inport
  assert_dv_per_sec : xbsIndex_r4/Assert  assert_type=on  type_source=Explicitly  gui_display_data_type=Fixed-point  arith_type=Unsigned  n_bits=32  bin_pt=0  preci_type=Single  exp_width=8  frac_width=24  assert_rate=off  rate_source=Explicitly  period=1  output_port=on  block_type=assert
  cast_gw : xbsIndex_r4/Convert  gui_display_data_type=Fixed-point  arith_type=Unsigned  n_bits=32  bin_pt=0  float_type=Single  exp_bits=8  fraction_bits=24  quantization=Truncate  overflow=Wrap  en=off  latency=1  pipeline=off  dbl_ovrd=off  block_type=convert
  io_delay : xbsIndex_r4/Delay  rst=off  infoeditControl=Selection of Reset will increase slice count due to use of real FFs and instead of SRLs  en=off  latency=0  reg_retiming=on  dbl_ovrd=off  block_type=delay
  reint1 : xbsIndex_r4/Reinterpret  force_arith_type=on  arith_type=Unsigned  force_bin_pt=on  bin_pt=0  block_type=reinterpret
  s_c_nbe_m32k_v9_reorder_status1_user_data_in : xbsIndex_r4/Gateway Out  inherit_from_input=off  hdl_port=on  rows=1  columns=1  UseAsDAC=off  DACChannel='1'  interface=None  automatic_assignment=on  address_offset=hex2dec('00')  intf_name=''  intf_description=''  timing_constraint=None  locs_specified=off  LOCs={}  io_standard={}  block_type=gatewayout
  sim_out : Terminator
  wires:
  io_delay/1 -> cast_gw/1
  cast_gw/1 -> s_c_nbe_m32k_v9_reorder_status1_user_data_in/1
  s_c_nbe_m32k_v9_reorder_status1_user_data_in/1 -> sim_out/1
  out_dv_per_sec/1 -> assert_dv_per_sec/1
  assert_dv_per_sec/1 -> reint1/1
  reint1/1 -> io_delay/1

== system s_c_nbe_m32k/rx_dest_ip ==
  out_reg : Inport
  assert_reg : xbsIndex_r4/Assert  assert_type=on  type_source=Explicitly  gui_display_data_type=Fixed-point  arith_type=Unsigned  n_bits=32  bin_pt=0  preci_type=Single  exp_width=8  frac_width=24  assert_rate=off  rate_source=Explicitly  period=1  output_port=on  block_type=assert
  cast_gw : xbsIndex_r4/Convert  gui_display_data_type=Fixed-point  arith_type=Unsigned  n_bits=32  bin_pt=0  float_type=Single  exp_bits=8  fraction_bits=24  quantization=Truncate  overflow=Wrap  en=off  latency=1  pipeline=off  dbl_ovrd=off  block_type=convert
  io_delay : xbsIndex_r4/Delay  rst=off  infoeditControl=Selection of Reset will increase slice count due to use of real FFs and instead of SRLs  en=off  latency=0  reg_retiming=on  dbl_ovrd=off  block_type=delay
  reint1 : xbsIndex_r4/Reinterpret  force_arith_type=on  arith_type=Unsigned  force_bin_pt=on  bin_pt=0  block_type=reinterpret
  s_c_nbe_m32k_v9_rx_dest_ip_user_data_in : xbsIndex_r4/Gateway Out  inherit_from_input=off  hdl_port=on  rows=1  columns=1  UseAsDAC=off  DACChannel='1'  interface=None  automatic_assignment=on  address_offset=hex2dec('00')  intf_name=''  intf_description=''  timing_constraint=None  locs_specified=off  LOCs={}  io_standard={}  block_type=gatewayout
  sim_out : Terminator
  wires:
  io_delay/1 -> cast_gw/1
  cast_gw/1 -> s_c_nbe_m32k_v9_rx_dest_ip_user_data_in/1
  s_c_nbe_m32k_v9_rx_dest_ip_user_data_in/1 -> sim_out/1
  out_reg/1 -> assert_reg/1
  assert_reg/1 -> reint1/1
  reint1/1 -> io_delay/1

== system s_c_nbe_m32k/snap_adc0 ==
  in_p0_d0 : Inport
  in_p0_d1 : Inport  Port=2
  in_p0_d2 : Inport  Port=3
  in_p0_d3 : Inport  Port=4
  in_p0_d4 : Inport  Port=5
  in_p0_d5 : Inport  Port=6
  in_p0_d6 : Inport  Port=7
  in_p0_d7 : Inport  Port=8
  in_dv : Inport  Port=9
  in_sync : Inport  Port=10
  we : Inport  Port=11
  trig : Inport  Port=12
  stop : Inport  Port=13
  extra_timestamp : Inport  Port=14
  assert_dv : xbsIndex_r4/Assert  assert_type=on  type_source=Explicitly  gui_display_data_type=Boolean  arith_type=Boolean  n_bits=1  bin_pt=0  preci_type=Single  exp_width=8  frac_width=24  assert_rate=off  rate_source=Explicitly  period=1  output_port=on  block_type=assert
  assert_p0_d{0..7} (8 alike) : xbsIndex_r4/Assert  assert_type=on  type_source=Explicitly  gui_display_data_type=Fixed-point  arith_type="Signed  (2's comp)"  n_bits=10  bin_pt=9  preci_type=Single  exp_width=8  frac_width=24  assert_rate=off  rate_source=Explicitly  period=1  output_port=on  block_type=assert
  assert_sync : xbsIndex_r4/Assert  assert_type=on  type_source=Explicitly  gui_display_data_type=Boolean  arith_type=Boolean  n_bits=1  bin_pt=0  preci_type=Single  exp_width=8  frac_width=24  assert_rate=off  rate_source=Explicitly  period=1  output_port=on  block_type=assert
  assextra_timestamp : xbsIndex_r4/Assert  assert_type=on  type_source=Explicitly  gui_display_data_type=Fixed-point  arith_type=Unsigned  n_bits=32  bin_pt=0  preci_type=Single  exp_width=8  frac_width=24  assert_rate=off  rate_source=Explicitly  period=1  output_port=on  block_type=assert
  buscreate : Subsystem  AncestorBlock=casper_library_flow_control/bus_create  mask(bus_create){inputNum=10}
      mask prompts: inputNum "Number of inputs:"
      mask init:
      | bus_create_init(gcb,...
      |     'inputNum', inputNum);
  extra_delay : Subsystem  AncestorBlock=casper_library_delays/pipeline  mask(pipeline){csp_latency=2}
      mask prompts: csp_latency "Latency"
      mask help:
      | An explicitly laid-out delay line to avoid mapping to SRL16s
      | for use in pipelining to help achieve timing closure.
      mask init:
      | pipeline_init(gcb,'latency',csp_latency);
      settings: AttributesFormatString=Latency = %<latency>
      mask Display:
      | port_label('input', 1, 'd');
      | port_label('output', 1, 'q');
      | disp(['Z^-', num2str(csp_latency)]);
  extracast : xbsIndex_r4/Convert  gui_display_data_type=Fixed-point  arith_type=Unsigned  n_bits=32  bin_pt=0  float_type=Single  exp_bits=8  fraction_bits=24  quantization=Truncate  overflow=Wrap  en=off  latency=1  pipeline=off  dbl_ovrd=off  block_type=convert
  extracreate : Subsystem  AncestorBlock=casper_library_flow_control/bus_create  mask(bus_create){inputNum=1}
      mask prompts: inputNum "Number of inputs:"
      mask init:
      | bus_create_init(gcb,...
      |     'inputNum', inputNum);
  io_delay : Subsystem  AncestorBlock=casper_library_delays/pipeline  mask(pipeline){csp_latency=2}
      mask prompts: csp_latency "Latency"
      mask help:
      | An explicitly laid-out delay line to avoid mapping to SRL16s
      | for use in pipelining to help achieve timing closure.
      mask init:
      | pipeline_init(gcb,'latency',csp_latency);
      settings: AttributesFormatString=Latency = %<latency>
      mask Display:
      | port_label('input', 1, 'd');
      | port_label('output', 1, 'q');
      | disp(['Z^-', num2str(csp_latency)]);
  ss : Subsystem  Tag=casper:snapshot  AncestorBlock=casper_library_scopes/snapshot  mask(snapshot){storage=bram, dram_dimm=2, dram_clock=250, nsamples=8, data_width=128, offset=off, circap=on, value=on, ext_arm=off, ext_circ=off, provide_outputs=off, use_dsp48=on}
      mask prompts: storage "Storage medium"; dram_dimm "DRAM dimm"; dram_clock "DRAM clock rate"; nsamples "Number of Samples (2^?)"; data_width "Data width"; offset "Start delay support"; circap "Circular capture support"; value "Extra value capture support"; ext_arm "External arm support"; ext_circ "External circular capture support"; provide_outputs "Provide outputs"; use_dsp48 "Use DSP48s to implement counters"
      mask help:
      | Standard snap block, but with the following optional extras;
      |  1) Optionally delay the fabric trigger by a user-specified number of valids.
      |  2) Capture continuously after a trigger until a stop pulse is received. Data is captured into BRAM continuously, with old data being overwritten until a stop command is received. Then stop capturing when memory is filled. This enables you to get some data before and some data after the stop pulse. Use the 'tr_en_cnt' register to determine where you are in your vector. 'Addr' register's MSb now indicates 'busy capturing'.
      |  3) Optionally capture a value on an input port to a register at the same time as the first data sample.
      |  4) Implement counters using DSP48Es to save resources.
      mask init:
      | snapshot_init(gcb, ...
      |     'storage', storage, ...
      |     'dram_dimm', dram_dimm, ...
      |     'dram_clock', dram_clock, ...
      |     'nsamples', nsamples, ...
      |     'data_width', data_width, ...
      |     'offset', offset, ...
      |     'circap', circap, ...
      |     'value', value, ...
      |     'ext_arm', ext_arm, ...
      |     'ext_circ', ext_circ, ...
      |     'provide_outputs', 'off', ...
      |     'use_dsp48', use_dsp48);
      settings: AttributesFormatString=|
      | 128 wide, 256 deep
      | debugID: 113545123
      mask TypeOptions storage: bram | dram
      mask Callback storage: snapshot_callback();
      mask TypeOptions dram_dimm: 1 | 2 | 3 | 4
      mask TypeOptions dram_clock: 200 | 250 | 266 | 300 | 333
      mask TypeOptions data_width: 8 | 16 | 32 | 64 | 128
  stop_delay : Subsystem  AncestorBlock=casper_library_delays/pipeline  mask(pipeline){csp_latency=2}
      mask prompts: csp_latency "Latency"
      mask help:
      | An explicitly laid-out delay line to avoid mapping to SRL16s
      | for use in pipelining to help achieve timing closure.
      mask init:
      | pipeline_init(gcb,'latency',csp_latency);
      settings: AttributesFormatString=Latency = %<latency>
      mask Display:
      | port_label('input', 1, 'd');
      | port_label('output', 1, 'q');
      | disp(['Z^-', num2str(csp_latency)]);
  trig_delay : Subsystem  AncestorBlock=casper_library_delays/pipeline  mask(pipeline){csp_latency=2}
      mask prompts: csp_latency "Latency"
      mask help:
      | An explicitly laid-out delay line to avoid mapping to SRL16s
      | for use in pipelining to help achieve timing closure.
      mask init:
      | pipeline_init(gcb,'latency',csp_latency);
      settings: AttributesFormatString=Latency = %<latency>
      mask Display:
      | port_label('input', 1, 'd');
      | port_label('output', 1, 'q');
      | disp(['Z^-', num2str(csp_latency)]);
  we_delay : Subsystem  AncestorBlock=casper_library_delays/pipeline  mask(pipeline){csp_latency=2}
      mask prompts: csp_latency "Latency"
      mask help:
      | An explicitly laid-out delay line to avoid mapping to SRL16s
      | for use in pipelining to help achieve timing closure.
      mask init:
      | pipeline_init(gcb,'latency',csp_latency);
      settings: AttributesFormatString=Latency = %<latency>
      mask Display:
      | port_label('input', 1, 'd');
      | port_label('output', 1, 'q');
      | disp(['Z^-', num2str(csp_latency)]);
  arm_out : Outport
  wires:
  ss/1(arm_out) -> arm_out/1
  buscreate/1(bus_out) -> io_delay/1(d)
  io_delay/1(q) -> ss/1(din)
  in_p0_d0/1 -> assert_p0_d0/1
  assert_p0_d0/1 -> buscreate/1(in1)
  in_p0_d1/1 -> assert_p0_d1/1
  assert_p0_d1/1 -> buscreate/2(in2)
  in_p0_d2/1 -> assert_p0_d2/1
  assert_p0_d2/1 -> buscreate/3(in3)
  in_p0_d3/1 -> assert_p0_d3/1
  assert_p0_d3/1 -> buscreate/4(in4)
  in_p0_d4/1 -> assert_p0_d4/1
  assert_p0_d4/1 -> buscreate/5(in5)
  in_p0_d5/1 -> assert_p0_d5/1
  assert_p0_d5/1 -> buscreate/6(in6)
  in_p0_d6/1 -> assert_p0_d6/1
  assert_p0_d6/1 -> buscreate/7(in7)
  in_p0_d7/1 -> assert_p0_d7/1
  assert_p0_d7/1 -> buscreate/8(in8)
  in_dv/1 -> assert_dv/1
  assert_dv/1 -> buscreate/9(in9)
  in_sync/1 -> assert_sync/1
  assert_sync/1 -> buscreate/10(in10)
  we/1 -> we_delay/1(d)
  we_delay/1(q) -> ss/2(we)
  trig/1 -> trig_delay/1(d)
  trig_delay/1(q) -> ss/3(trig)
  stop/1 -> stop_delay/1(d)
  stop_delay/1(q) -> ss/4(stop)
  extracreate/1(bus_out) -> extra_delay/1(d)
  extra_delay/1(q) -> extracast/1
  extracast/1 -> ss/5(vin)
  extra_timestamp/1 -> assextra_timestamp/1
  assextra_timestamp/1 -> extracreate/1(in1)
